simulink model "PMSM_Simulation_2025a"  (R2025a)
settings: Solver=FixedStepDiscrete  StartTime=0.0  StopTime=10  FixedStep=0.00005/200  RelTol=1e-3
values from neighbouring files (symbols this model uses):
  MC_DCurrLopKi_CFG = 0.008293758    [PMSM_MC_Data_2025a.sldd]
  MC_DCurrLopKp_CFG = 0.0870848    [PMSM_MC_Data_2025a.sldd]
  MC_MotModeDebug_CFG = 255.0    [PMSM_MC_Data_2025a.sldd]
  MC_POLE_NUM_CFG = 7.0    [PMSM_MC_Data_2025a.sldd]
  MC_QCurrLopKi_CFG = 0.008293758    [PMSM_MC_Data_2025a.sldd]
  MC_QCurrLopKp_CFG = 0.0870848    [PMSM_MC_Data_2025a.sldd]
  MC_SpdLopKi_CFG = 1.0E-5    [PMSM_MC_Data_2025a.sldd]
  MC_SpdLopKp_CFG = 0.002    [PMSM_MC_Data_2025a.sldd]
undefined symbols (not defined in the file or in its folder): Ls, magnitude, Rs
libraries: simulink x28, slpidlib x6, spsDCVoltageSourceLib x1, spsPermanentMagnetSynchronousMachineLib x1, spsUniversalBridgeLib x1, sps_lib x1
(part 2 of 3)

== system PMSM_Simulation_2025a/PMSM_MC/MC_HighFrqTask/FOC/SensorLessAlgorithm ==
  note: MotorSpdRef用于
      | 方向极性判定使用
  MotorSpdRef : Inport
  Ialpha : Inport  Port=2
  Ibeta : Inport  Port=3
  Ualpha : Inport  Port=4
  Ubeta : Inport  Port=5
  Compare To Constant : simulink/Logic and Bit Operations/Compare To Constant  relop===  const=0  OutDataTypeStr=boolean
  Compare To Constant1 : simulink/Logic and Bit Operations/Compare To Constant  relop===  const=1  OutDataTypeStr=boolean
  Compare To Constant2 : simulink/Logic and Bit Operations/Compare To Constant  relop===  const=2  OutDataTypeStr=boolean
  Compare To Constant3 : simulink/Logic and Bit Operations/Compare To Constant  relop===  const=3  OutDataTypeStr=boolean
  Constant : Constant  Value=uint8(3)
  FluxObs+PLL : Subsystem
  Luenberger+PLL : Subsystem
  Merge : Merge  Inputs=4
  Merge1 : Merge  Inputs=4
  SMO+Artan : Subsystem
  SMO+PLL : Subsystem
  Thetae_Est : Outport
  We_Est : Outport  Port=2
  wires:
  MotorSpdRef/1 -> SMO+Artan/1(MotorSpdRef), Luenberger+PLL/1(MotorSpdRef), FluxObs+PLL/1(MotorSpdRef), SMO+PLL/1(MotorSpdRef)
  Ialpha/1 -> SMO+Artan/2(Ialpha), Luenberger+PLL/2(Ialpha), FluxObs+PLL/2(Ialpha), SMO+PLL/2(Ialpha)
  Ibeta/1 -> Luenberger+PLL/3(Ibeta), FluxObs+PLL/3(Ibeta), SMO+PLL/3(Ibeta), SMO+Artan/3(Ibeta)
  Ualpha/1 -> Luenberger+PLL/4(Ualpha), FluxObs+PLL/4(Ualpha), SMO+PLL/4(Ualpha), SMO+Artan/4(Ualpha)
  Ubeta/1 -> Luenberger+PLL/5(Ubeta), FluxObs+PLL/5(Ubeta), SMO+PLL/5(Ubeta), SMO+Artan/5(Ubeta)
  Constant/1 -> Compare To Constant3/1, Compare To Constant2/1, Compare To Constant1/1, Compare To Constant/1
  Compare To Constant/1 -> SMO+Artan/Enable
  Compare To Constant1/1 -> SMO+PLL/Enable
  Compare To Constant2/1 -> FluxObs+PLL/Enable
  SMO+Artan/1(Thetae_Est) -> Merge/1
  SMO+PLL/1(Thetae_Est) -> Merge/2
  FluxObs+PLL/1(Thetae_Est) -> Merge/3
  Luenberger+PLL/1(Thetae_Est) -> Merge/4
  SMO+Artan/2(We_Est) -> Merge1/1
  SMO+PLL/2(We_Est) -> Merge1/2
  FluxObs+PLL/2(We_Est) -> Merge1/3
  Luenberger+PLL/2(We_Est) -> Merge1/4
  Merge1/1 -> We_Est/1
  Merge/1 -> Thetae_Est/1
  Compare To Constant3/1 -> Luenberger+PLL/Enable

== system PMSM_Simulation_2025a/PMSM_MC/MC_HighFrqTask/OpenLopMod/AngleNormalization ==
  note: 用于将观测器估算的输入角度归一化到[0 2pi]的角度输出
  Theta : Inport
  Abs : Abs  SaturateOnIntegerOverflow=off
  Add : Sum  Inputs=+-
  Compare To Zero : simulink/Logic and Bit Operations/Compare To Zero  relop=>=  OutDataTypeStr=boolean
  Constant : Constant  Value=single(6.28)
  Constant1 : Constant  Value=single(6.28)
  Constant2 : Constant  Value=single(6.28)
  Mod : Math  Operator=mod
  Mod1 : Math  Operator=mod
  Switch : Switch  Criteria=u2 ~= 0  SaturateOnIntegerOverflow=off  InputSameDT=off
  ThetaNorm : Outport
  wires:
  Theta/1 -> Abs/1, Mod/1, Compare To Zero/1
  Compare To Zero/1 -> Switch/2
  Constant/1 -> Mod/2
  Mod/1 -> Switch/1
  Abs/1 -> Mod1/1
  Constant1/1 -> Mod1/2
  Add/1 -> Switch/3
  Mod1/1 -> Add/2
  Constant2/1 -> Add/1
  Switch/1 -> ThetaNorm/1

== system PMSM_Simulation_2025a/PMSM_MC/MC_LowFrqTask/MotSpdCal/LPF ==
  In : Inport
  TiCon : Inport  Port=2
  Add : Sum  Inputs=+-
  Add1 : Sum
  Constant : Constant  Value=single(1)
  Delay : Delay  DelayLength=1  InitialConditionSource=Input port
      settings: InputPortMap=u0,p4
  Product : Product
  Product1 : Product
  out : Outport
  wires:
  In/1 -> Delay/2, Product/1
  TiCon/1 -> Add/2, Product/2
  Add/1 -> Product1/1
  Constant/1 -> Add/1
  Product/1 -> Add1/1
  Product1/1 -> Add1/2
  Add1/1 -> Delay/1, out/1
  Delay/1 -> Product1/2

== system PMSM_Simulation_2025a/PMSM_MC/MC_LowFrqTask/MotSpdCal/LPF1 ==
  In : Inport
  TiCon : Inport  Port=2
  Add : Sum  Inputs=+-
  Add1 : Sum
  Constant : Constant  Value=single(1)
  Delay : Delay  DelayLength=1  InitialConditionSource=Input port
      settings: InputPortMap=u0,p4
  Product : Product
  Product1 : Product
  out : Outport
  wires:
  In/1 -> Delay/2, Product/1
  TiCon/1 -> Add/2, Product/2
  Add/1 -> Product1/1
  Constant/1 -> Add/1
  Product/1 -> Add1/1
  Product1/1 -> Add1/2
  Add1/1 -> Delay/1, out/1
  Delay/1 -> Product1/2

== system PMSM_Simulation_2025a/PMSM_MC/MC_HighFrqTask/ElecAngleCal/AngleCal/If Action Subsystem ==
  Ecode_PhyVal : Inport
  Action Port : ActionPort  ActionPortLabel=if(u1 == 1)
  Constant : Constant  Value=MC_POLE_NUM_CFG
  Constant1 : Constant  Value=int32(16384)
  Constant2 : Constant  Value=int32(16384)
  Constant3 : Constant  Value=single(6.28)
  Data Type Conversion : DataTypeConversion  OutDataTypeStr=single  SaturateOnIntegerOverflow=off  RndMeth=Floor
  Data Type Conversion1 : DataTypeConversion  OutDataTypeStr=single  SaturateOnIntegerOverflow=off  RndMeth=Floor
  Data Type Conversion2 : DataTypeConversion  OutDataTypeStr=single  SaturateOnIntegerOverflow=off  RndMeth=Floor
  Divide : Product  Inputs=*/
  Mod : Math  Operator=mod
  Mux : Mux  Inputs=2
  Product : Product
  Product1 : Product
  Out1 : Outport
  wires:
  Ecode_PhyVal/1 -> Mod/1
  Constant1/1 -> Mod/2
  Mod/1 -> Data Type Conversion/1
  Data Type Conversion/1 -> Divide/1
  Constant2/1 -> Divide/2
  Divide/1 -> Product/1
  Constant3/1 -> Product/2
  Constant/1 -> Data Type Conversion1/1
  Data Type Conversion1/1 -> Product1/2
  Product/1 -> Product1/1, Mux/1
  Product1/1 -> Data Type Conversion2/1
  Data Type Conversion2/1 -> Mux/2
  Mux/1 -> Out1/1

== system PMSM_Simulation_2025a/PMSM_MC/MC_HighFrqTask/ElecAngleCal/AngleCal/If Action Subsystem1 ==
  Ecode_PhyVal : Inport
  Action Port : ActionPort  ActionPortLabel=elseif(u1 == -1)
  Constant : Constant  Value=MC_POLE_NUM_CFG
  Constant1 : Constant  Value=int32(16384)
  Constant2 : Constant  Value=int32(16384)
  Constant3 : Constant  Value=single(6.28)
  Data Type Conversion : DataTypeConversion  OutDataTypeStr=single  SaturateOnIntegerOverflow=off  RndMeth=Floor
  Data Type Conversion1 : DataTypeConversion  OutDataTypeStr=single  SaturateOnIntegerOverflow=off  RndMeth=Floor
  Data Type Conversion2 : DataTypeConversion  OutDataTypeStr=single  SaturateOnIntegerOverflow=off  RndMeth=Floor
  Data Type Conversion3 : DataTypeConversion  OutDataTypeStr=int32  SaturateOnIntegerOverflow=off  RndMeth=Floor
  Divide : Product  Inputs=*/
  Gain : Gain  Gain=-1
  Gain1 : Gain  Gain=-1
  Mod : Math  Operator=mod
  Mux : Mux  Inputs=2
  Product : Product
  Product1 : Product
  Out1 : Outport
  wires:
  Constant1/1 -> Mod/2
  Mod/1 -> Data Type Conversion/1
  Constant2/1 -> Divide/2
  Constant3/1 -> Product/2
  Data Type Conversion2/1 -> Mux/2
  Product/1 -> Product1/1, Mux/1
  Divide/1 -> Product/1
  Constant/1 -> Data Type Conversion1/1
  Data Type Conversion/1 -> Divide/1
  Product1/1 -> Data Type Conversion2/1
  Data Type Conversion1/1 -> Product1/2
  Ecode_PhyVal/1 -> Gain/1
  Gain/1 -> Data Type Conversion3/1
  Data Type Conversion3/1 -> Mod/1
  Mux/1 -> Gain1/1
  Gain1/1 -> Out1/1

== system PMSM_Simulation_2025a/PMSM_MC/MC_HighFrqTask/ElecAngleCal/AngleCal/If Action Subsystem2 ==
  Action Port : ActionPort  ActionPortLabel=else
  Constant : Constant  Value=single(0)
  Constant1 : Constant  Value=single(0)
  Mux : Mux  Inputs=2
  Out1 : Outport
  wires:
  Constant/1 -> Mux/1
  Constant1/1 -> Mux/2
  Mux/1 -> Out1/1

== system PMSM_Simulation_2025a/PMSM_MC/MC_HighFrqTask/FOC/SVPWM/SevenSegSVPWM ==
  Uα : Inport
  Uβ : Inport  Port=2
  VBus : Inport  Port=3
  Demux : Demux  Outputs=3
  SectorCaculate : Subsystem
  T1T2Caculate : Subsystem
  TcmCaculate : Subsystem
  Tpwm : Constant  Value=single(1)
  XYZCaculate : Subsystem
  UVoltage_PWM : Outport
  VVoltage_PWM : Outport  Port=2
  WVoltage_PWM : Outport  Port=3
  wires:
  Uα/1 -> SectorCaculate/1(Ualpha), XYZCaculate/1(Ualpha)
  Uβ/1 -> XYZCaculate/2(Ubeta), SectorCaculate/2(Ubeta)
  VBus/1 -> XYZCaculate/3(Udc)
  Tpwm/1 -> TcmCaculate/4(Tpwm), T1T2Caculate/3(Tpwm), XYZCaculate/4(Ts)
  SectorCaculate/1(N) -> TcmCaculate/1(N), T1T2Caculate/1(N)
  XYZCaculate/1(XYZ) -> T1T2Caculate/2(XYZ)
  T1T2Caculate/1(T1) -> TcmCaculate/2(T1)
  T1T2Caculate/2(T2) -> TcmCaculate/3(T2)
  TcmCaculate/1(Tcm1 Tcm2 Tcm3) -> Demux/1
  Demux/1 -> UVoltage_PWM/1
  Demux/2 -> VVoltage_PWM/1
  Demux/3 -> WVoltage_PWM/1

== system PMSM_Simulation_2025a/PMSM_MC/MC_HighFrqTask/FOC/SensorLessAlgorithm/FluxObs+PLL ==
  MotorSpdRef : Inport
  Ialpha : Inport  Port=2
  Ibeta : Inport  Port=3
  Ualpha : Inport  Port=4
  Ubeta : Inport  Port=5
  Enable : EnablePort
  FluxObs : Subsystem
  PLL : Subsystem
  Thetae_Est : Outport
  We_Est : Outport  Port=2
  wires:
  Ubeta/1 -> FluxObs/4(Ubeta)
  Ualpha/1 -> FluxObs/3(Ualpha)
  Ialpha/1 -> FluxObs/1(Ialpha)
  Ibeta/1 -> FluxObs/2(Ibeta)
  PLL/1(Thetae_Est) -> Thetae_Est/1
  PLL/2(We_Est) -> We_Est/1
  FluxObs/2(Flux_beta) -> PLL/3(Flux_beta)
  FluxObs/1(Flux_alpha) -> PLL/2(Flux_alpha)
  MotorSpdRef/1 -> PLL/1(MotorSpdRef)

== system PMSM_Simulation_2025a/PMSM_MC/MC_HighFrqTask/FOC/SensorLessAlgorithm/Luenberger+PLL ==
  MotorSpdRef : Inport
  Ialpha : Inport  Port=2
  Ibeta : Inport  Port=3
  Ualpha : Inport  Port=4
  Ubeta : Inport  Port=5
  Enable : EnablePort
  Delay : Delay  DelayLength=1
  Luenberger : Subsystem
  PLL : Subsystem
  Thetae_Est : Outport
  We_Est : Outport  Port=2
  wires:
  MotorSpdRef/1 -> PLL/1(MotorSpdRef)
  Luenberger/1(AlphaE) -> PLL/2(AlphaE)
  Luenberger/2(BetaE) -> PLL/3(BetaE)
  PLL/2(We_Est) -> Delay/1, We_Est/1
  PLL/1(Thetae_Est) -> Thetae_Est/1
  Ibeta/1 -> Luenberger/2(Ibeta)
  Ialpha/1 -> Luenberger/1(Ialpha)
  Ualpha/1 -> Luenberger/3(Ualpha)
  Ubeta/1 -> Luenberger/4(Ubeta)
  Delay/1 -> Luenberger/5(We)

== system PMSM_Simulation_2025a/PMSM_MC/MC_HighFrqTask/FOC/SensorLessAlgorithm/SMO+Artan ==
  MotorSpdRef : Inport
  Ialpha : Inport  Port=2
  Ibeta : Inport  Port=3
  Ualpha : Inport  Port=4
  Ubeta : Inport  Port=5
  Enable : EnablePort
  Artan : Subsystem
  SMO : Subsystem
  Thetae_Est : Outport
  We_Est : Outport  Port=2
  wires:
  Ialpha/1 -> SMO/1(Ialpha)
  Ibeta/1 -> SMO/2(Ibeta)
  Ualpha/1 -> SMO/3(Ualpha)
  Ubeta/1 -> SMO/4(Ubeta)
  MotorSpdRef/1 -> Artan/1(MotorSpdRef)
  SMO/1(AlphaE) -> Artan/2(AlphaE)
  SMO/2(BetaE) -> Artan/3(BetaE)
  Artan/2(We_Est) -> We_Est/1
  Artan/1(Thetae_Est) -> Thetae_Est/1

== system PMSM_Simulation_2025a/PMSM_MC/MC_HighFrqTask/FOC/SensorLessAlgorithm/SMO+PLL ==
  MotorSpdRef : Inport
  Ialpha : Inport  Port=2
  Ibeta : Inport  Port=3
  Ualpha : Inport  Port=4
  Ubeta : Inport  Port=5
  Enable : EnablePort
  PLL : Subsystem
  SMO : Subsystem
  Thetae_Est : Outport
  We_Est : Outport  Port=2
  wires:
  MotorSpdRef/1 -> PLL/1(MotorSpdRef)
  SMO/1(AlphaE) -> PLL/2(AlphaE)
  SMO/2(BetaE) -> PLL/3(BetaE)
  PLL/2(We_Est) -> We_Est/1
  PLL/1(Thetae_Est) -> Thetae_Est/1
  Ibeta/1 -> SMO/2(Ibeta)
  Ialpha/1 -> SMO/1(Ialpha)
  Ualpha/1 -> SMO/3(Ualpha)
  Ubeta/1 -> SMO/4(Ubeta)

== system PMSM_Simulation_2025a/PMSM_MC/MC_HighFrqTask/FOC/SVPWM/SevenSegSVPWM/SectorCaculate ==
  Ualpha : Inport
  Ubeta : Inport  Port=2
  A : Fcn  Expr=u[2]
  Add : Sum  Inputs=+++
  B : Fcn  Expr=u(1)*sqrt(3/4)-0.5*u[2]
  C : Fcn  Expr=-u[1]*sqrt(3/4)-u[2]*0.5
  Constant : Constant  Value=uint8(1)
  Constant1 : Constant  Value=uint8(0)
  Data Type Conversion : DataTypeConversion  OutDataTypeStr=uint8  SaturateOnIntegerOverflow=off  RndMeth=Floor
  Gain : Gain  Gain=2
  Gain1 : Gain  Gain=4
  Mux : Mux  Inputs=2
  Switch : Switch  Criteria=u2 > Threshold  SaturateOnIntegerOverflow=off  InputSameDT=off
  Switch1 : Switch  Criteria=u2 > Threshold  SaturateOnIntegerOverflow=off  InputSameDT=off
  Switch2 : Switch  Criteria=u2 > Threshold  SaturateOnIntegerOverflow=off  InputSameDT=off
  N : Outport
  wires:
  Ualpha/1 -> Mux/1
  Ubeta/1 -> Mux/2
  Mux/1 -> C/1, A/1, B/1
  A/1 -> Switch/2
  B/1 -> Switch1/2
  C/1 -> Switch2/2
  Constant/1 -> Switch/1, Switch2/1, Switch1/1
  Constant1/1 -> Switch/3, Switch1/3, Switch2/3
  Switch2/1 -> Gain1/1
  Switch1/1 -> Gain/1
  Gain/1 -> Add/2
  Gain1/1 -> Add/3
  Switch/1 -> Add/1
  Add/1 -> Data Type Conversion/1
  Data Type Conversion/1 -> N/1

== system PMSM_Simulation_2025a/PMSM_MC/MC_HighFrqTask/FOC/SVPWM/SevenSegSVPWM/T1T2Caculate ==
  N : Inport
  XYZ : Inport  Port=2
  Tpwm : Inport  Port=3
  Abs : Abs  SaturateOnIntegerOverflow=off
  Abs1 : Abs  SaturateOnIntegerOverflow=off
  Demux : Demux  Outputs=3
  Fcn : Fcn  Expr=u(1)*u(3)/(u(1)+u(2))
  Fcn1 : Fcn  Expr=u(2)*u(3)/(u(1)+u(2))
  Fcn2 : Fcn  Expr=u(3)-u(2)-u(1)
  Gain : Gain  Gain=-1
  Gain1 : Gain  Gain=-1
  Gain2 : Gain  Gain=-1
  Multiport Switch : MultiPortSwitch  Inputs=6  DiagnosticForDefault=None  SaturateOnIntegerOverflow=off  InputSameDT=off
  Multiport Switch1 : MultiPortSwitch  Inputs=6  DiagnosticForDefault=None  SaturateOnIntegerOverflow=off  InputSameDT=off
  Mux : Mux  Inputs=3
  Switch : Switch  SaturateOnIntegerOverflow=off  InputSameDT=off
  Switch1 : Switch  SaturateOnIntegerOverflow=off  InputSameDT=off
  T1 : Outport
  T2 : Outport  Port=2
  wires:
  N/1 -> Multiport Switch/1, Multiport Switch1/1
  XYZ/1 -> Demux/1
  Demux/1 -> Gain/1, Multiport Switch/6, Multiport Switch1/4
  Demux/2 -> Gain1/1, Multiport Switch/3, Multiport Switch1/2
  Demux/3 -> Gain2/1, Multiport Switch1/5, Multiport Switch/2
  Gain/1 -> Multiport Switch1/3, Multiport Switch/5
  Gain2/1 -> Multiport Switch1/7, Multiport Switch/4
  Gain1/1 -> Multiport Switch/7, Multiport Switch1/6
  Multiport Switch/1 -> Switch/1, Mux/1  "T1"
  Multiport Switch1/1 -> Switch1/1, Mux/2  "T2"
  Tpwm/1 -> Mux/3
  Mux/1 -> Fcn1/1, Fcn/1, Fcn2/1
  Fcn/1 -> Switch/3
  Fcn1/1 -> Switch1/3
  Fcn2/1 -> Switch1/2, Switch/2
  Switch/1 -> Abs/1
  Abs/1 -> T1/1
  Switch1/1 -> Abs1/1
  Abs1/1 -> T2/1

== system PMSM_Simulation_2025a/PMSM_MC/MC_HighFrqTask/FOC/SVPWM/SevenSegSVPWM/TcmCaculate ==
  N : Inport
  T1 : Inport  Port=2
  T2 : Inport  Port=3
  Tpwm : Inport  Port=4
  Fcn : Fcn  Expr=(u(3)+u(1)+u(2))/2
  Fcn1 : Fcn  Expr=(u(3)-u(1)+u(2))/2
  Fcn2 : Fcn  Expr=(u(3)-u(1)-u(2))/2
  Multiport Switch : MultiPortSwitch  Inputs=6  DiagnosticForDefault=None  SaturateOnIntegerOverflow=off  InputSameDT=off
  Multiport Switch1 : MultiPortSwitch  Inputs=6  DiagnosticForDefault=None  SaturateOnIntegerOverflow=off  InputSameDT=off
  Multiport Switch2 : MultiPortSwitch  Inputs=6  DiagnosticForDefault=None  SaturateOnIntegerOverflow=off  InputSameDT=off
  Mux : Mux  Inputs=3
  Mux1 : Mux  Inputs=3
  Tcm1 Tcm2 Tcm3 : Outport
  wires:
  Mux/1 -> Tcm1 Tcm2 Tcm3/1
  T2/1 -> Mux1/2
  T1/1 -> Mux1/1
  Tpwm/1 -> Mux1/3
  Mux1/1 -> Fcn/1, Fcn2/1, Fcn1/1
  N/1 -> Multiport Switch2/1, Multiport Switch1/1, Multiport Switch/1
  Fcn1/1 -> Multiport Switch1/4, Multiport Switch/7, Multiport Switch/2, Multiport Switch1/5, Multiport Switch2/6, Multiport Switch2/3
  Fcn/1 -> Multiport Switch1/6, Multiport Switch2/7, Multiport Switch2/5, Multiport Switch/4, Multiport Switch/3, Multiport Switch1/2
  Fcn2/1 -> Multiport Switch1/7, Multiport Switch/6, Multiport Switch/5, Multiport Switch1/3, Multiport Switch2/4, Multiport Switch2/2
  Multiport Switch/1 -> Mux/1
  Multiport Switch1/1 -> Mux/2
  Multiport Switch2/1 -> Mux/3

== system PMSM_Simulation_2025a/PMSM_MC/MC_HighFrqTask/FOC/SVPWM/SevenSegSVPWM/XYZCaculate ==
  Ualpha : Inport
  Ubeta : Inport  Port=2
  Udc : Inport  Port=3
  Ts : Inport  Port=4
  Add : Sum
  Add1 : Sum  Inputs=+-
  Fcn : Fcn  Expr=1/u
  Gain : Gain  Gain=3/2
  Gain1 : Gain  Gain=sqrt(3)
  Gain2 : Gain  Gain=sqrt(3)/2
  Mux : Mux  Inputs=3
  Product{,1..3} (4 alike) : Product
  XYZ : Outport
  wires:
  Ualpha/1 -> Gain/1
  Ubeta/1 -> Gain2/1, Gain1/1
  Gain/1 -> Add/2, Add1/2
  Gain1/1 -> Product/1
  Gain2/1 -> Add1/1, Add/1
  Ts/1 -> Product3/1
  Product3/1 -> Product1/2, Product/2, Product2/2
  Add/1 -> Product1/1
  Udc/1 -> Fcn/1
  Fcn/1 -> Product3/2
  Add1/1 -> Product2/1
  Product1/1 -> Mux/2
  Product2/1 -> Mux/3
  Product/1 -> Mux/1
  Mux/1 -> XYZ/1

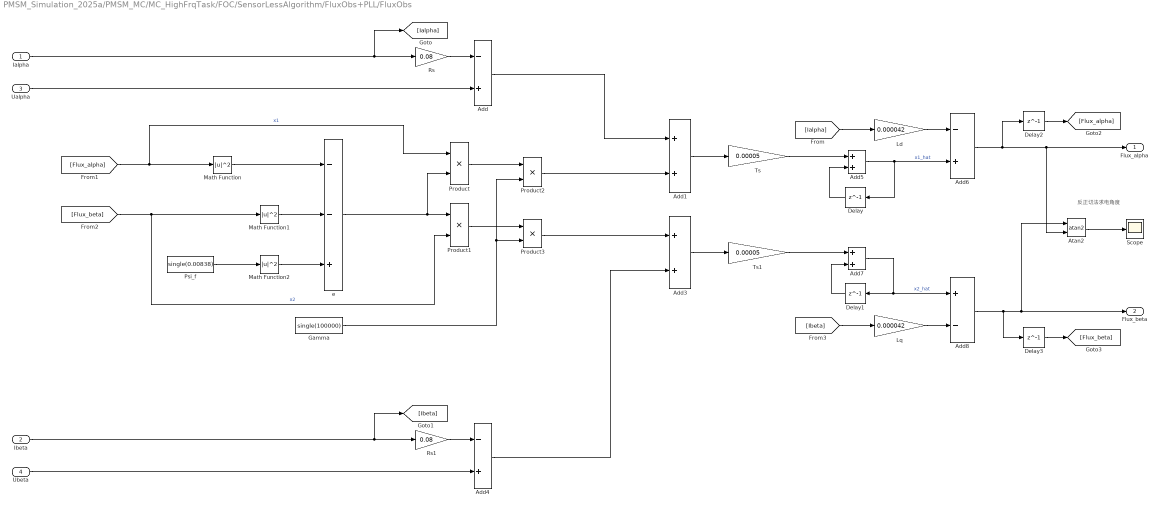
== system PMSM_Simulation_2025a/PMSM_MC/MC_HighFrqTask/FOC/SensorLessAlgorithm/FluxObs+PLL/FluxObs ==
  note: 反正切法求电角度
  Ialpha : Inport
  Ibeta : Inport  Port=2
  Ualpha : Inport  Port=3
  Ubeta : Inport  Port=4
  Add : Sum  Inputs=-+
  Add{1,3,5,7} (4 alike) : Sum
  Add4 : Sum  Inputs=-+
  Add6 : Sum  Inputs=-+
  Add8 : Sum  Inputs=+-
  Atan2 : Trigonometry  Operator=atan2
  Delay{,1..3} (4 alike) : Delay  DelayLength=1
  Gamma : Constant  Value=single(100000)
  Ld : Gain  Gain=0.000042
  Lq : Gain  Gain=0.000042
  Math Function : Math  Operator=magnitude^2
  Math Function1 : Math  Operator=magnitude^2
  Math Function2 : Math  Operator=magnitude^2
  Product{,1..3} (4 alike) : Product
  Psi_f : Constant  Value=single(0.00838)
  Rs : Gain  Gain=0.08
  Rs1 : Gain  Gain=0.08
  Scope : Scope
      settings: ActiveDisplayYMinimum=-3.9256648123264313  ActiveDisplayYMaximum=3.9258014261722565  DataLoggingVariableName=ScopeData8
  Ts : Gain  Gain=0.00005
  Ts1 : Gain  Gain=0.00005
  e : Sum  Inputs=--+
  Flux_alpha : Outport
  Flux_beta : Outport  Port=2
  wires:
  Ialpha/1 -> [Ialpha], Rs/1
  Rs/1 -> Add/1
  Ualpha/1 -> Add/2
  Add/1 -> Add1/1
  [Flux_alpha] -> Product/1, Math Function/1  "x1"
  Math Function/1 -> e/1
  [Flux_beta] -> Product1/2, Math Function1/1  "x2"
  Math Function1/1 -> e/2
  Math Function2/1 -> e/3
  Psi_f/1 -> Math Function2/1
  e/1 -> Product1/1, Product/2
  Product/1 -> Product2/1
  Product1/1 -> Product3/1
  Gamma/1 -> Product2/2, Product3/2
  Product2/1 -> Add1/2
  Product3/1 -> Add3/1
  Ubeta/1 -> Add4/2
  Ibeta/1 -> [Ibeta], Rs1/1
  Rs1/1 -> Add4/1
  Add4/1 -> Add3/2
  Add1/1 -> Ts/1
  Add3/1 -> Ts1/1
  Ts/1 -> Add5/1
  [Ialpha] -> Ld/1
  Ld/1 -> Add6/1
  Add5/1 -> Delay/1, Add6/2  "x1_hat"
  Delay/1 -> Add5/2
  Ts1/1 -> Add7/1
  Add7/1 -> Add8/1, Delay1/1  "x2_hat"
  Delay1/1 -> Add7/2
  Lq/1 -> Add8/2
  [Ibeta] -> Lq/1
  Add6/1 -> Delay2/1, Atan2/2, Flux_alpha/1
  Add8/1 -> Delay3/1, Atan2/1, Flux_beta/1
  Delay2/1 -> [Flux_alpha]
  Delay3/1 -> [Flux_beta]
  Atan2/1 -> Scope/1

== system PMSM_Simulation_2025a/PMSM_MC/MC_HighFrqTask/FOC/SensorLessAlgorithm/FluxObs+PLL/PLL ==
  MotorSpdRef : Inport
  Flux_alpha : Inport  Port=2
  Flux_beta : Inport  Port=3
  Add : Sum
  Constant : Constant  Value=single(52000)
  Constant1 : Constant  Value=single(0.0085)
  Constant4 : Constant  Value=single(40)
  Constant5 : Constant  Value=single(2*pi)
  Cos : Trigonometry  Operator=cos
  Delay : Delay  DelayLength=1
  Gain : Gain  Gain=0.00005
  LPF : Subsystem
  Mod : Math  Operator=mod
  PI_Out : Scope  NumInputPorts=2
      settings: ActiveDisplayYMinimum=-82.912358522415147  ActiveDisplayYMaximum=519.20902562141418  DataLoggingVariableName=ScopeData11
  PLL_PI : slpidlib/PID Controller  Controller=PI  Form=Parallel  TimeDomain=Discrete-time  UseExternalTs=off  SampleTime=-1  IntegratorMethod=Forward Euler  FilterMethod=Forward Euler  ControllerParametersSource=external  P=1  I=1  UseKiTs=on  D=0  UseExternalDerivativeSource=off  N=100  UseFilter=on  TunerSelectOption=Transfer Function Based (PID Tuner App)  InitialConditionSource=internal  InitialConditionForIntegrator=0  InitialConditionForFilter=0  DifferentiatorICPrevScaledInput=0  ExternalReset=none  TrackingMode=off  Kt=1  LimitOutput=off  SatLimitsSource=internal  UpperSaturationLimit=inf  LowerSaturationLimit=-inf  LinearizeAsGain=off  AntiWindupMode=none  Kb=1  LimitIntegrator=off  UpperIntegratorSaturationLimit=8000  LowerIntegratorSaturationLimit=-8000  POutMin=[]  POutMax=[]  IOutMin=[]  IOutMax=[]  DOutMin=[]  DOutMax=[]  NOutMin=[]  NOutMax=[]  SumOutMin=[]  SumOutMax=[]  SaturationOutMin=[]  SaturationOutMax=[]  PParamMin=[]  PParamMax=[]  IParamMin=[]  IParamMax=[]  DParamMin=[]  DParamMax=[]  NParamMin=[]  NParamMax=[]  KbParamMin=[]  KbParamMax=[]  KtParamMin=[]  KtParamMax=[]  KbOutMin=[]  KbOutMax=[]  KtOutMin=[]  KtOutMax=[]  IntegratorOutMin=[]  IntegratorOutMax=[]  FilterOutMin=[]  FilterOutMax=[]  SumI1OutMin=[]  SumI1OutMax=[]  SumI2OutMin=[]  SumI2OutMax=[]  SumI3OutMin=[]  SumI3OutMax=[]  SumI4OutMin=[]  SumI4OutMax=[]  SumDOutMin=[]  SumDOutMax=[]  DifferentiatorOutMin=[]  DifferentiatorOutMax=[]  FilterDiffOutCoefMin=[]  FilterDiffOutCoefMax=[]  ReciprocalOutMin=[]  ReciprocalOutMax=[]  SumDenOutMin=[]  SumDenOutMax=[]  SumNumOutMin=[]  SumNumOutMax=[]  DivideOutMin=[]  DivideOutMax=[]  UdiffTsProdOutMin=[]  UdiffTsProdOutMax=[]  NTsProdOutMin=[]  NTsProdOutMax=[]  UintegralTsProdOutMin=[]  UintegralTsProdOutMax=[]  UngainTsProdOutMin=[]  UngainTsProdOutMax=[]  ClampingZeroOutDataTypeStr=Inherit: Inherit via back propagation  ClampingZeroOutMin=[]  ClampingZeroOutMax=[]  FilterDenConstantOutDataTypeStr=Inherit: Inherit via back propagation  FilterDenConstantOutMin=[]  FilterDenConstantOutMax=[]  PCopyOutDataTypeStr=Inherit: Inherit via back propagation  PCopyOutMin=[]  PCopyOutMax=[]  NCopyOutDataTypeStr=Inherit: Inherit via back propagation  NCopyOutMin=[]  NCopyOutMax=[]  IntegratorContinuousStateAttributes=''  IntegratorStateMustResolveToSignalObject=off  IntegratorRTWStateStorageClass=Auto  FilterContinuousStateAttributes=''  FilterStateMustResolveToSignalObject=off  FilterRTWStateStorageClass=Auto  ParallelPVariant=ExternalParameters  IdealPVariant=Disabled  IVariant=ExternalParameters  DVariant=Disabled  IntegratorVariant=Discrete  SatVariant=Disabled  AWVariant=Passthrough  PCopyVariant=Disabled  TRVariant=Disabled  FdbkBlocksVariant=Forward  IdealPFdbkVariant=Disabled  SatFdbkVariant=Disabled  DerivativeFilterVariant=Disabled  NVariant=Disabled  NCopyVariant=Disabled_SignalSpec  FilterICVariant=Disabled  IntegratorICVariant=InternalICs  ExternalResetVariant=Disabled  TRSumVariant=Passthrough  SumFdbkVariant=Disabled  SumVariant=Sum_PI  TsampFilterVariant=InternalTs  TsampNgainVariant=Passthrough  TsampIntegralVariant=Disabled_SignalSpec  ExternalSaturationOutDataTypeStr=Inherit: Same as second input  DerivativeSourceVariant=Disabled  PreIntVariant=InternalPreInt
      settings: LibrarySourceBlock=simulink/Discrete/Discrete PID Controller
  Product : Product
  Product2 : Product
  Sin : Trigonometry
  err : Sum  Inputs=-+
  erro : Scope
      settings: ActiveDisplayYMinimum=-0.010186117957346141  ActiveDisplayYMaximum=0.0015268082497641442  DataLoggingVariableName=ScopeData10
  Thetae_Est : Outport
  We_Est : Outport  Port=2
  wires:
  Delay/1 -> Add/2, Cos/1, Sin/1
  Mod/1 -> Thetae_Est/1, Delay/1
  Constant5/1 -> Mod/2
  Add/1 -> Mod/1
  Gain/1 -> Add/1
  PLL_PI/1 -> PI_Out/1, LPF/1(In), Gain/1
  Constant4/1 -> PLL_PI/3
  Constant/1 -> PLL_PI/2
  Cos/1 -> Product2/1
  Sin/1 -> Product/1
  LPF/1(out) -> PI_Out/2, We_Est/1
  Constant1/1 -> LPF/2(TiCon)
  Flux_alpha/1 -> Product/2
  Flux_beta/1 -> Product2/2
  Product/1 -> err/1
  Product2/1 -> err/2
  err/1 -> erro/1, PLL_PI/1

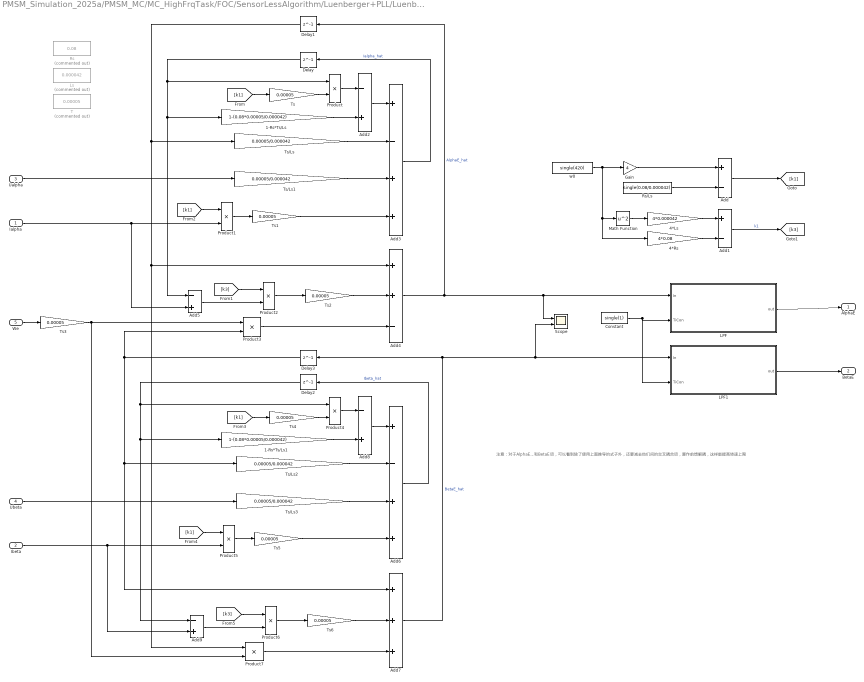
== system PMSM_Simulation_2025a/PMSM_MC/MC_HighFrqTask/FOC/SensorLessAlgorithm/Luenberger+PLL/Luenberger ==
  note: 注意：对于AlphaE和BetaE项，可以看到除了使用上面推导的式子外，还要减去他们间的交叉耦合项，算作前馈解耦，这样能提高转速上限
  Ialpha : Inport
  Ibeta : Inport  Port=2
  Ualpha : Inport  Port=3
  Ubeta : Inport  Port=4
  We : Inport  Port=5
  1-Rs*Ts/Ls : Gain  Gain=1-(0.08*0.00005/0.000042)
  1-Rs*Ts/Ls1 : Gain  Gain=1-(0.08*0.00005/0.000042)
  4*Ls : Gain  Gain=4*0.000042
  4*Rs : Gain  Gain=4*0.08
  Add : Sum  Inputs=+-
  Add1 : Sum  Inputs=+-
  Add{2,5,8..9} (4 alike) : Sum  Inputs=-+
  Add3 : Sum  Inputs=+-++
  Add4 : Sum  Inputs=++-
  Add6 : Sum  Inputs=+-++
  Add7 : Sum  Inputs=+++
  Constant : Constant  Value=single(1)
  Delay{,1..3} (4 alike) : Delay  DelayLength=1
  Gain : Gain  Gain=4
  LPF : Subsystem
  LPF1 : Subsystem
  Ls : Constant  Commented=on  Value=0.000042
  Math Function : Math  Operator=square
  Product{,1..7} (8 alike) : Product
  Rs : Constant  Commented=on  Value=0.08
  Rs/Ls : Constant  Value=single(0.08/0.000042)
  Scope : Scope  NumInputPorts=2
      settings: ActiveDisplayYMinimum=-21.479682207107544  ActiveDisplayYMaximum=21.825211763381958  DataLoggingVariableName=ScopeData18
  T : Constant  Commented=on  Value=0.00005
  Ts{,1..6} (7 alike) : Gain  Gain=0.00005
  Ts/Ls{,1..3} (4 alike) : Gain  Gain=0.00005/0.000042
  w0 : Constant  Value=single(420)
  AlphaE : Outport
  BetaE : Outport  Port=2
  wires:
  w0/1 -> 4*Rs/1, Math Function/1, Gain/1
  Add/1 -> [k1]
  Rs/Ls/1 -> Add/2
  Gain/1 -> Add/1
  4*Ls/1 -> Add1/1
  4*Rs/1 -> Add1/2
  Math Function/1 -> 4*Ls/1
  Add1/1 -> [k3]  "k1"
  [k1] -> Ts/1
  Ts/1 -> Product/2
  Product/1 -> Add2/1
  1-Rs*Ts/Ls/1 -> Add2/2
  Ts/Ls/1 -> Add3/2
  Add2/1 -> Add3/1
  Ts/Ls1/1 -> Add3/3
  [k1] -> Product1/1
  Product1/1 -> Ts1/1
  Ts1/1 -> Add3/4
  Ialpha/1 -> Add5/2, Product1/2
  Ualpha/1 -> Ts/Ls1/1
  Add3/1 -> Delay/1  "Ialpha_hat"
  Delay/1 -> Add5/1, 1-Rs*Ts/Ls/1, Product/1
  Add4/1 -> Scope/1, LPF/1(In), Delay1/1  "AlphaE_hat"
  Delay1/1 -> Product7/1, Add4/1, Ts/Ls/1
  Ts2/1 -> Add4/2
  Product2/1 -> Ts2/1
  [k3] -> Product2/1
  Add5/1 -> Product2/2
  Constant/1 -> LPF1/2(TiCon), LPF/2(TiCon)
  LPF1/1(out) -> BetaE/1
  LPF/1(out) -> AlphaE/1
  We/1 -> Ts3/1
  Product3/1 -> Add4/3
  Add6/1 -> Delay2/1  "Ibeta_hat"
  Product4/1 -> Add8/1
  Delay2/1 -> Product4/1, 1-Rs*Ts/Ls1/1, Add9/1
  1-Rs*Ts/Ls1/1 -> Add8/2
  Ts4/1 -> Product4/2
  [k1] -> Ts4/1
  Add8/1 -> Add6/1
  [k1] -> Product5/1
  Ibeta/1 -> Product5/2, Add9/2
  Delay3/1 -> Ts/Ls2/1, Add7/1, Product3/2
  Ubeta/1 -> Ts/Ls3/1
  Product5/1 -> Ts5/1
  Ts/Ls3/1 -> Add6/3
  Ts5/1 -> Add6/4
  Ts/Ls2/1 -> Add6/2
  Product7/1 -> Add7/3
  Product6/1 -> Ts6/1
  [k3] -> Product6/1
  Add9/1 -> Product6/2
  Ts3/1 -> Product3/1, Product7/2
  Ts6/1 -> Add7/2
  Add7/1 -> Scope/2, LPF1/1(In), Delay3/1  "BetaE_hat"

== system PMSM_Simulation_2025a/PMSM_MC/MC_HighFrqTask/FOC/SensorLessAlgorithm/Luenberger+PLL/PLL ==
  note: 根据误差式子设定来设定反电动势
      | 符号确保使得PLL形成负反馈
  MotorSpdRef : Inport
  AlphaE : Inport  Port=2
  BetaE : Inport  Port=3
  Add : Sum
  Compare To Zero1 : simulink/Logic and Bit Operations/Compare To Zero  relop=>=  OutDataTypeStr=boolean
  Constant : Constant  Value=single(200)
  Constant1 : Constant  Value=single(0.0085)
  Constant2 : Constant  Value=single(-1)
  Constant3 : Constant  Value=single(1)
  Constant4 : Constant  Value=single(2)
  Constant5 : Constant  Value=single(2*pi)
  Cos : Trigonometry  Operator=cos
  Delay : Delay  DelayLength=1
  Gain : Gain  Gain=0.00005
  LPF : Subsystem
  Mod : Math  Operator=mod
  PLL_PI : slpidlib/PID Controller  Controller=PI  Form=Parallel  TimeDomain=Discrete-time  UseExternalTs=off  SampleTime=-1  IntegratorMethod=Forward Euler  FilterMethod=Forward Euler  ControllerParametersSource=external  P=1  I=1  UseKiTs=on  D=0  UseExternalDerivativeSource=off  N=100  UseFilter=on  TunerSelectOption=Transfer Function Based (PID Tuner App)  InitialConditionSource=internal  InitialConditionForIntegrator=0  InitialConditionForFilter=0  DifferentiatorICPrevScaledInput=0  ExternalReset=none  TrackingMode=off  Kt=1  LimitOutput=off  SatLimitsSource=internal  UpperSaturationLimit=inf  LowerSaturationLimit=-inf  LinearizeAsGain=off  AntiWindupMode=none  Kb=1  LimitIntegrator=off  UpperIntegratorSaturationLimit=inf  LowerIntegratorSaturationLimit=-inf  POutMin=[]  POutMax=[]  IOutMin=[]  IOutMax=[]  DOutMin=[]  DOutMax=[]  NOutMin=[]  NOutMax=[]  SumOutMin=[]  SumOutMax=[]  SaturationOutMin=[]  SaturationOutMax=[]  PParamMin=[]  PParamMax=[]  IParamMin=[]  IParamMax=[]  DParamMin=[]  DParamMax=[]  NParamMin=[]  NParamMax=[]  KbParamMin=[]  KbParamMax=[]  KtParamMin=[]  KtParamMax=[]  KbOutMin=[]  KbOutMax=[]  KtOutMin=[]  KtOutMax=[]  IntegratorOutMin=[]  IntegratorOutMax=[]  FilterOutMin=[]  FilterOutMax=[]  SumI1OutMin=[]  SumI1OutMax=[]  SumI2OutMin=[]  SumI2OutMax=[]  SumI3OutMin=[]  SumI3OutMax=[]  SumI4OutMin=[]  SumI4OutMax=[]  SumDOutMin=[]  SumDOutMax=[]  DifferentiatorOutMin=[]  DifferentiatorOutMax=[]  FilterDiffOutCoefMin=[]  FilterDiffOutCoefMax=[]  ReciprocalOutMin=[]  ReciprocalOutMax=[]  SumDenOutMin=[]  SumDenOutMax=[]  SumNumOutMin=[]  SumNumOutMax=[]  DivideOutMin=[]  DivideOutMax=[]  UdiffTsProdOutMin=[]  UdiffTsProdOutMax=[]  NTsProdOutMin=[]  NTsProdOutMax=[]  UintegralTsProdOutMin=[]  UintegralTsProdOutMax=[]  UngainTsProdOutMin=[]  UngainTsProdOutMax=[]  ClampingZeroOutDataTypeStr=Inherit: Inherit via back propagation  ClampingZeroOutMin=[]  ClampingZeroOutMax=[]  FilterDenConstantOutDataTypeStr=Inherit: Inherit via back propagation  FilterDenConstantOutMin=[]  FilterDenConstantOutMax=[]  PCopyOutDataTypeStr=Inherit: Inherit via back propagation  PCopyOutMin=[]  PCopyOutMax=[]  NCopyOutDataTypeStr=Inherit: Inherit via back propagation  NCopyOutMin=[]  NCopyOutMax=[]  IntegratorContinuousStateAttributes=''  IntegratorStateMustResolveToSignalObject=off  IntegratorRTWStateStorageClass=Auto  FilterContinuousStateAttributes=''  FilterStateMustResolveToSignalObject=off  FilterRTWStateStorageClass=Auto  ParallelPVariant=ExternalParameters  IdealPVariant=Disabled  IVariant=ExternalParameters  DVariant=Disabled  IntegratorVariant=Discrete  SatVariant=Disabled  AWVariant=Passthrough  PCopyVariant=Disabled  TRVariant=Disabled  FdbkBlocksVariant=Forward  IdealPFdbkVariant=Disabled  SatFdbkVariant=Disabled  DerivativeFilterVariant=Disabled  NVariant=Disabled  NCopyVariant=Disabled_SignalSpec  FilterICVariant=Disabled  IntegratorICVariant=InternalICs  ExternalResetVariant=Disabled  TRSumVariant=Passthrough  SumFdbkVariant=Disabled  SumVariant=Sum_PI  TsampFilterVariant=InternalTs  TsampNgainVariant=Passthrough  TsampIntegralVariant=Disabled_SignalSpec  ExternalSaturationOutDataTypeStr=Inherit: Same as second input  DerivativeSourceVariant=Disabled  PreIntVariant=InternalPreInt
      settings: LibrarySourceBlock=simulink/Discrete/Discrete PID Controller
  Product{,1..3} (4 alike) : Product
  Sin : Trigonometry
  Switch1 : Switch  Criteria=u2 ~= 0  SaturateOnIntegerOverflow=off  InputSameDT=off
  err : Sum
  Thetae_Est : Outport
  We_Est : Outport  Port=2
  wires:
  Gain/1 -> Add/1
  Mod/1 -> Delay/1, Thetae_Est/1
  AlphaE/1 -> Product/2
  Constant4/1 -> PLL_PI/3
  Product/1 -> Product1/1
  Constant3/1 -> Switch1/3
  Constant5/1 -> Mod/2
  Switch1/1 -> Product3/2, Product1/2
  Product3/1 -> err/2
  Delay/1 -> Cos/1, Sin/1, Add/2
  err/1 -> PLL_PI/1
  Compare To Zero1/1 -> Switch1/2
  Constant2/1 -> Switch1/1
  PLL_PI/1 -> Gain/1, LPF/1(In)
  Cos/1 -> Product/1
  Sin/1 -> Product2/1
  MotorSpdRef/1 -> Compare To Zero1/1
  BetaE/1 -> Product2/2
  Constant/1 -> PLL_PI/2
  LPF/1(out) -> We_Est/1
  Product1/1 -> err/1
  Constant1/1 -> LPF/2(TiCon)
  Product2/1 -> Product3/1
  Add/1 -> Mod/1

== system PMSM_Simulation_2025a/PMSM_MC/MC_HighFrqTask/FOC/SensorLessAlgorithm/SMO+Artan/Artan ==
  note: 速度计算
      | 包含过零处计算处理
  note: 根据速度期望设定来设定反电动势符号
  note: 得使用atan2，而不是atan，
      | 因为atan函数无法判断象限
      | 输出的值是[-PI,PI]
  note: 将角度归一化到[0,2PI]
  MotorSpdRef : Inport
  AlphaE : Inport  Port=2
  BetaE : Inport  Port=3
  Add : Sum  Inputs=+-
  Compare To Zero : simulink/Logic and Bit Operations/Compare To Zero  relop=>=  OutDataTypeStr=boolean
  Constant : Constant  Value=single(2*pi)
  Constant1 : Constant  Value=single(0.01)
  Data Type Conversion : DataTypeConversion  OutDataTypeStr=single  SaturateOnIntegerOverflow=off  RndMeth=Floor
  Gain : Gain  Gain=-1
  Gain1 : Gain  Gain=-1
  LPF : Subsystem
  Product : Product
  Product1 : Product
  Scope : Scope  NumInputPorts=2
      settings: ActiveDisplayYMinimum=-82058.83984375  ActiveDisplayYMaximum=82039.71484375  DataLoggingVariableName=ScopeData13
  Scope1 : Scope
      settings: ActiveDisplayYMinimum=-0.7852557301521299  ActiveDisplayYMaximum=7.0673015713691711  DataLoggingVariableName=ScopeData15
  Sign : Signum
  Sin : Trigonometry  Operator=atan2
  Switch : Switch  Criteria=u2 ~= 0  SaturateOnIntegerOverflow=off  InputSameDT=off
  WeCal : Subsystem
  Thetae_Est : Outport
  We_Est : Outport  Port=2
  wires:
  MotorSpdRef/1 -> Sign/1
  Sign/1 -> Data Type Conversion/1
  AlphaE/1 -> Product/1
  BetaE/1 -> Product1/1
  Data Type Conversion/1 -> Product1/2, Product/2
  Product/1 -> Sin/1
  Product1/1 -> Sin/2
  Sin/1 -> Gain/1
  Gain/1 -> Gain1/1, Switch/1, Compare To Zero/1
  Compare To Zero/1 -> Switch/2
  Gain1/1 -> Add/2
  Constant/1 -> Add/1
  Add/1 -> Switch/3
  Switch/1 -> WeCal/1(ArTan_theta_est), Scope1/1, Thetae_Est/1
  Constant1/1 -> LPF/2(TiCon)
  WeCal/1(We) -> Scope/1, LPF/1(In)
  LPF/1(out) -> Scope/2, We_Est/1

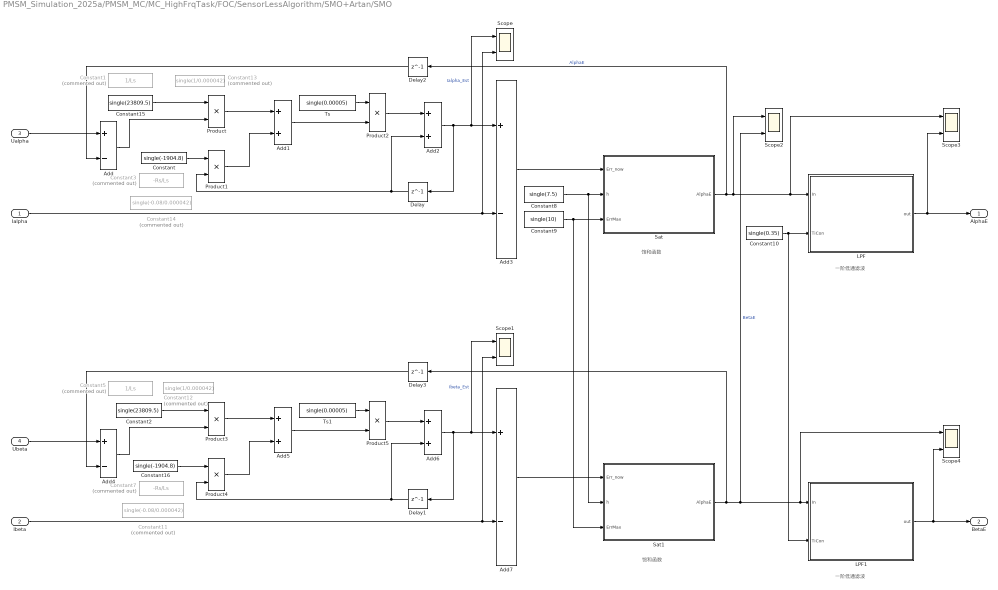
== system PMSM_Simulation_2025a/PMSM_MC/MC_HighFrqTask/FOC/SensorLessAlgorithm/SMO+Artan/SMO ==
  note: 一阶低通滤波
  note: 饱和函数
  note: 饱和函数
  note: 一阶低通滤波
  Ialpha : Inport
  Ibeta : Inport  Port=2
  Ualpha : Inport  Port=3
  Ubeta : Inport  Port=4
  Add{,3..4,7} (4 alike) : Sum  Inputs=+-
  Add{1..2,5..6} (4 alike) : Sum
  Constant : Constant  Value=single(-1904.8)
  Constant1 : Constant  Commented=on  Value=1/Ls
  Constant10 : Constant  Value=single(0.35)
  Constant11 : Constant  Commented=on  Value=single(-0.08/0.000042)
  Constant12 : Constant  Commented=on  Value=single(1/0.000042)
  Constant13 : Constant  Commented=on  Value=single(1/0.000042)
  Constant14 : Constant  Commented=on  Value=single(-0.08/0.000042)
  Constant15 : Constant  Value=single(23809.5)
  Constant16 : Constant  Value=single(-1904.8)
  Constant2 : Constant  Value=single(23809.5)
  Constant3 : Constant  Commented=on  Value=-Rs/Ls
  Constant5 : Constant  Commented=on  Value=1/Ls
  Constant7 : Constant  Commented=on  Value=-Rs/Ls
  Constant8 : Constant  Value=single(7.5)
  Constant9 : Constant  Value=single(10)
  Delay{,1..3} (4 alike) : Delay  DelayLength=1
  LPF : Subsystem
  LPF1 : Subsystem
  Product{,1..5} (6 alike) : Product
  Sat : Subsystem
  Sat1 : Subsystem
  Scope{,1..4} (5 alike) : Scope  NumInputPorts=2
      Scope settings: ActiveDisplayYMinimum=-20.242838406954043  ActiveDisplayYMaximum=19.683035350457061  DataLoggingVariableName=ScopeData2
      Scope1 settings: DataLoggingVariableName=ScopeData3
      Scope2 settings: ActiveDisplayYMinimum=-6.6872910357846731  ActiveDisplayYMaximum=6.6852858453807853  DataLoggingVariableName=ScopeData4
      Scope3 settings: DataLoggingVariableName=ScopeData5
      Scope4 settings: ActiveDisplayYMinimum=-7.4362883952418741  ActiveDisplayYMaximum=7.436170963264396  DataLoggingVariableName=ScopeData6
  Ts : Constant  Value=single(0.00005)
  Ts1 : Constant  Value=single(0.00005)
  AlphaE : Outport
  BetaE : Outport  Port=2
  wires:
  Ualpha/1 -> Add/1
  Constant15/1 -> Product/1
  Add/1 -> Product/2
  Product/1 -> Add1/1
  Constant/1 -> Product1/1
  Product1/1 -> Add1/2
  Add1/1 -> Product2/2
  Ts/1 -> Product2/1
  Product2/1 -> Add2/1
  Add2/1 -> Delay/1, Scope/1, Add3/1  "Ialpha_Est"
  Delay/1 -> Add2/2, Product1/2
  Ialpha/1 -> Scope/2, Add3/2
  Product5/1 -> Add6/1
  Delay1/1 -> Add6/2, Product4/2
  Product3/1 -> Add5/1
  Ibeta/1 -> Scope1/2, Add7/2
  Ts1/1 -> Product5/1
  Add4/1 -> Product3/2
  Constant2/1 -> Product3/1
  Product4/1 -> Add5/2
  Constant16/1 -> Product4/1
  Add5/1 -> Product5/2
  Add6/1 -> Delay1/1, Scope1/1, Add7/1  "Ibeta_Est"
  Ubeta/1 -> Add4/1
  Add3/1 -> Sat/1(Err_now)
  Constant8/1 -> Sat1/2(h), Sat/2(h)
  Constant9/1 -> Sat1/3(ErrMax), Sat/3(ErrMax)
  Add7/1 -> Sat1/1(Err_now)
  Sat/1(AlphaE) -> Scope2/1, Scope3/1, LPF/1(In), Delay2/1  "AlphaE"
  Delay2/1 -> Add/2
  Sat1/1(AlphaE) -> Scope2/2, Scope4/1, LPF1/1(In), Delay3/1  "BetaE"
  Delay3/1 -> Add4/2
  Constant10/1 -> LPF/2(TiCon), LPF1/2(TiCon)
  LPF/1(out) -> Scope3/2, AlphaE/1
  LPF1/1(out) -> Scope4/2, BetaE/1

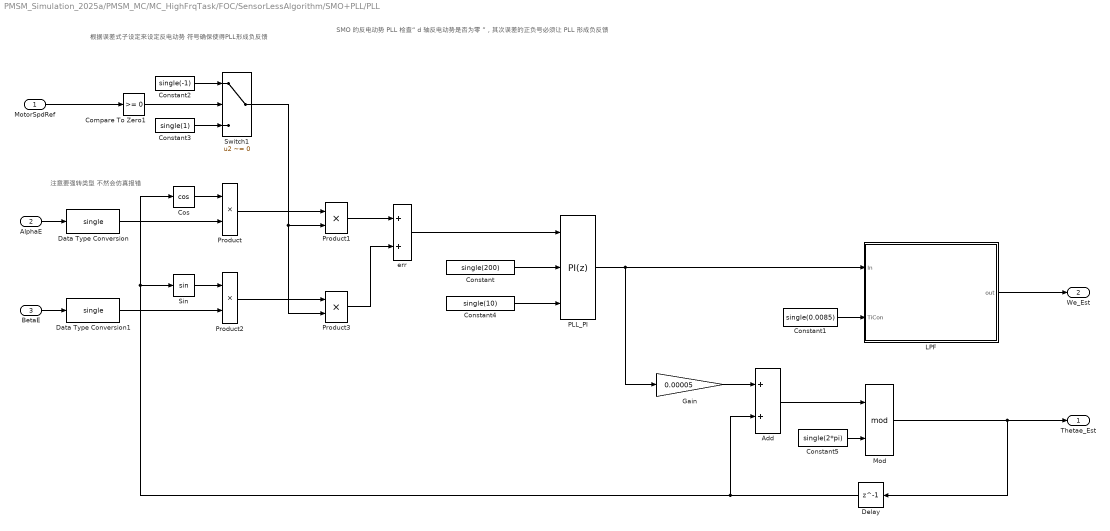
== system PMSM_Simulation_2025a/PMSM_MC/MC_HighFrqTask/FOC/SensorLessAlgorithm/SMO+PLL/PLL ==
  note: SMO 的反电动势 PLL 检查“ d 轴反电动势是否为零 ”，其次误差的正负号必须让 PLL 形成负反馈
  note: 注意要强转类型
      | 不然会仿真报错
  note: 根据误差式子设定来设定反电动势
      | 符号确保使得PLL形成负反馈
  MotorSpdRef : Inport
  AlphaE : Inport  Port=2
  BetaE : Inport  Port=3
  Add : Sum
  Compare To Zero1 : simulink/Logic and Bit Operations/Compare To Zero  relop=>=  OutDataTypeStr=boolean
  Constant : Constant  Value=single(200)
  Constant1 : Constant  Value=single(0.0085)
  Constant2 : Constant  Value=single(-1)
  Constant3 : Constant  Value=single(1)
  Constant4 : Constant  Value=single(10)
  Constant5 : Constant  Value=single(2*pi)
  Cos : Trigonometry  Operator=cos
  Data Type Conversion : DataTypeConversion  OutDataTypeStr=single  SaturateOnIntegerOverflow=off  RndMeth=Floor
  Data Type Conversion1 : DataTypeConversion  OutDataTypeStr=single  SaturateOnIntegerOverflow=off  RndMeth=Floor
  Delay : Delay  DelayLength=1
  Gain : Gain  Gain=0.00005
  LPF : Subsystem
  Mod : Math  Operator=mod
  PLL_PI : slpidlib/PID Controller  Controller=PI  Form=Parallel  TimeDomain=Discrete-time  UseExternalTs=off  SampleTime=-1  IntegratorMethod=Forward Euler  FilterMethod=Forward Euler  ControllerParametersSource=external  P=1  I=1  UseKiTs=on  D=0  UseExternalDerivativeSource=off  N=100  UseFilter=on  TunerSelectOption=Transfer Function Based (PID Tuner App)  InitialConditionSource=internal  InitialConditionForIntegrator=0  InitialConditionForFilter=0  DifferentiatorICPrevScaledInput=0  ExternalReset=none  TrackingMode=off  Kt=1  LimitOutput=off  SatLimitsSource=internal  UpperSaturationLimit=inf  LowerSaturationLimit=-inf  LinearizeAsGain=off  AntiWindupMode=none  Kb=1  LimitIntegrator=off  UpperIntegratorSaturationLimit=inf  LowerIntegratorSaturationLimit=-inf  POutMin=[]  POutMax=[]  IOutMin=[]  IOutMax=[]  DOutMin=[]  DOutMax=[]  NOutMin=[]  NOutMax=[]  SumOutMin=[]  SumOutMax=[]  SaturationOutMin=[]  SaturationOutMax=[]  PParamMin=[]  PParamMax=[]  IParamMin=[]  IParamMax=[]  DParamMin=[]  DParamMax=[]  NParamMin=[]  NParamMax=[]  KbParamMin=[]  KbParamMax=[]  KtParamMin=[]  KtParamMax=[]  KbOutMin=[]  KbOutMax=[]  KtOutMin=[]  KtOutMax=[]  IntegratorOutMin=[]  IntegratorOutMax=[]  FilterOutMin=[]  FilterOutMax=[]  SumI1OutMin=[]  SumI1OutMax=[]  SumI2OutMin=[]  SumI2OutMax=[]  SumI3OutMin=[]  SumI3OutMax=[]  SumI4OutMin=[]  SumI4OutMax=[]  SumDOutMin=[]  SumDOutMax=[]  DifferentiatorOutMin=[]  DifferentiatorOutMax=[]  FilterDiffOutCoefMin=[]  FilterDiffOutCoefMax=[]  ReciprocalOutMin=[]  ReciprocalOutMax=[]  SumDenOutMin=[]  SumDenOutMax=[]  SumNumOutMin=[]  SumNumOutMax=[]  DivideOutMin=[]  DivideOutMax=[]  UdiffTsProdOutMin=[]  UdiffTsProdOutMax=[]  NTsProdOutMin=[]  NTsProdOutMax=[]  UintegralTsProdOutMin=[]  UintegralTsProdOutMax=[]  UngainTsProdOutMin=[]  UngainTsProdOutMax=[]  ClampingZeroOutDataTypeStr=Inherit: Inherit via back propagation  ClampingZeroOutMin=[]  ClampingZeroOutMax=[]  FilterDenConstantOutDataTypeStr=Inherit: Inherit via back propagation  FilterDenConstantOutMin=[]  FilterDenConstantOutMax=[]  PCopyOutDataTypeStr=Inherit: Inherit via back propagation  PCopyOutMin=[]  PCopyOutMax=[]  NCopyOutDataTypeStr=Inherit: Inherit via back propagation  NCopyOutMin=[]  NCopyOutMax=[]  IntegratorContinuousStateAttributes=''  IntegratorStateMustResolveToSignalObject=off  IntegratorRTWStateStorageClass=Auto  FilterContinuousStateAttributes=''  FilterStateMustResolveToSignalObject=off  FilterRTWStateStorageClass=Auto  ParallelPVariant=ExternalParameters  IdealPVariant=Disabled  IVariant=ExternalParameters  DVariant=Disabled  IntegratorVariant=Discrete  SatVariant=Disabled  AWVariant=Passthrough  PCopyVariant=Disabled  TRVariant=Disabled  FdbkBlocksVariant=Forward  IdealPFdbkVariant=Disabled  SatFdbkVariant=Disabled  DerivativeFilterVariant=Disabled  NVariant=Disabled  NCopyVariant=Disabled_SignalSpec  FilterICVariant=Disabled  IntegratorICVariant=InternalICs  ExternalResetVariant=Disabled  TRSumVariant=Passthrough  SumFdbkVariant=Disabled  SumVariant=Sum_PI  TsampFilterVariant=InternalTs  TsampNgainVariant=Passthrough  TsampIntegralVariant=Disabled_SignalSpec  ExternalSaturationOutDataTypeStr=Inherit: Same as second input  DerivativeSourceVariant=Disabled  PreIntVariant=InternalPreInt
      settings: LibrarySourceBlock=simulink/Discrete/Discrete PID Controller
  Product{,1..3} (4 alike) : Product
  Sin : Trigonometry
  Switch1 : Switch  Criteria=u2 ~= 0  SaturateOnIntegerOverflow=off  InputSameDT=off
  err : Sum
  Thetae_Est : Outport
  We_Est : Outport  Port=2
  wires:
  MotorSpdRef/1 -> Compare To Zero1/1
  Compare To Zero1/1 -> Switch1/2
  Constant1/1 -> LPF/2(TiCon)
  LPF/1(out) -> We_Est/1
  Constant2/1 -> Switch1/1
  Constant3/1 -> Switch1/3
  Cos/1 -> Product/1
  Product/1 -> Product1/1
  Switch1/1 -> Product3/2, Product1/2
  Sin/1 -> Product2/1
  Product2/1 -> Product3/1
  Product1/1 -> err/1
  Product3/1 -> err/2
  err/1 -> PLL_PI/1
  Constant/1 -> PLL_PI/2
  Constant4/1 -> PLL_PI/3
  PLL_PI/1 -> Gain/1, LPF/1(In)
  Gain/1 -> Add/1
  Add/1 -> Mod/1
  Constant5/1 -> Mod/2
  Mod/1 -> Delay/1, Thetae_Est/1
  Delay/1 -> Cos/1, Sin/1, Add/2
  BetaE/1 -> Data Type Conversion1/1
  AlphaE/1 -> Data Type Conversion/1
  Data Type Conversion/1 -> Product/2
  Data Type Conversion1/1 -> Product2/2

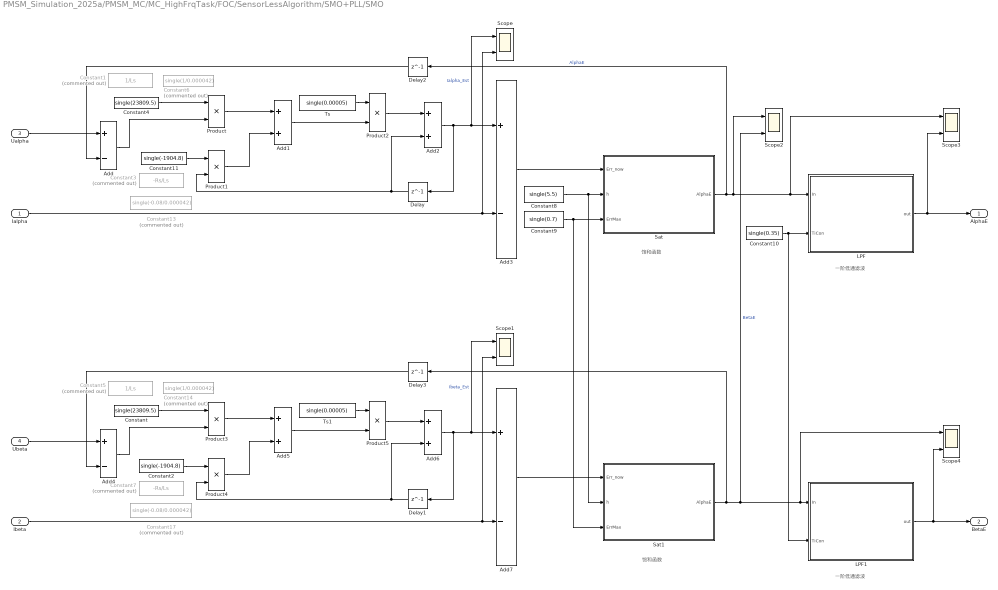
== system PMSM_Simulation_2025a/PMSM_MC/MC_HighFrqTask/FOC/SensorLessAlgorithm/SMO+PLL/SMO ==
  note: 一阶低通滤波
  note: 饱和函数
  note: 饱和函数
  note: 一阶低通滤波
  Ialpha : Inport
  Ibeta : Inport  Port=2
  Ualpha : Inport  Port=3
  Ubeta : Inport  Port=4
  Add{,3..4,7} (4 alike) : Sum  Inputs=+-
  Add{1..2,5..6} (4 alike) : Sum
  Constant : Constant  Value=single(23809.5)
  Constant1 : Constant  Commented=on  Value=1/Ls
  Constant10 : Constant  Value=single(0.35)
  Constant11 : Constant  Value=single(-1904.8)
  Constant13 : Constant  Commented=on  Value=single(-0.08/0.000042)
  Constant14 : Constant  Commented=on  Value=single(1/0.000042)
  Constant17 : Constant  Commented=on  Value=single(-0.08/0.000042)
  Constant2 : Constant  Value=single(-1904.8)
  Constant3 : Constant  Commented=on  Value=-Rs/Ls
  Constant4 : Constant  Value=single(23809.5)
  Constant5 : Constant  Commented=on  Value=1/Ls
  Constant6 : Constant  Commented=on  Value=single(1/0.000042)
  Constant7 : Constant  Commented=on  Value=-Rs/Ls
  Constant8 : Constant  Value=single(5.5)
  Constant9 : Constant  Value=single(0.7)
  Delay{,1..3} (4 alike) : Delay  DelayLength=1
  LPF : Subsystem
  LPF1 : Subsystem
  Product{,1..5} (6 alike) : Product
  Sat : Subsystem
  Sat1 : Subsystem
  Scope{,1..4} (5 alike) : Scope  NumInputPorts=2
      Scope settings: ActiveDisplayYMinimum=-11.265603890227075  ActiveDisplayYMaximum=11.401321085088421  DataLoggingVariableName=ScopeData2
      Scope1 settings: DataLoggingVariableName=ScopeData3
      Scope2 settings: ActiveDisplayYMinimum=-6.875  ActiveDisplayYMaximum=6.875  DataLoggingVariableName=ScopeData4
      Scope3 settings: DataLoggingVariableName=ScopeData5
      Scope4 settings: DataLoggingVariableName=ScopeData6
  Ts : Constant  Value=single(0.00005)
  Ts1 : Constant  Value=single(0.00005)
  AlphaE : Outport
  BetaE : Outport  Port=2
  wires:
  Ualpha/1 -> Add/1
  Constant4/1 -> Product/1
  Add/1 -> Product/2
  Product/1 -> Add1/1
  Constant11/1 -> Product1/1
  Product1/1 -> Add1/2
  Add1/1 -> Product2/2
  Ts/1 -> Product2/1
  Product2/1 -> Add2/1
  Add2/1 -> Delay/1, Scope/1, Add3/1  "Ialpha_Est"
  Delay/1 -> Add2/2, Product1/2
  Ialpha/1 -> Scope/2, Add3/2
  Product5/1 -> Add6/1
  Delay1/1 -> Add6/2, Product4/2
  Product3/1 -> Add5/1
  Ibeta/1 -> Scope1/2, Add7/2
  Ts1/1 -> Product5/1
  Add4/1 -> Product3/2
  Constant/1 -> Product3/1
  Product4/1 -> Add5/2
  Constant2/1 -> Product4/1
  Add5/1 -> Product5/2
  Add6/1 -> Delay1/1, Scope1/1, Add7/1  "Ibeta_Est"
  Ubeta/1 -> Add4/1
  Add3/1 -> Sat/1(Err_now)
  Constant8/1 -> Sat1/2(h), Sat/2(h)
  Constant9/1 -> Sat1/3(ErrMax), Sat/3(ErrMax)
  Add7/1 -> Sat1/1(Err_now)
  Sat/1(AlphaE) -> Scope2/1, Scope3/1, LPF/1(In), Delay2/1  "AlphaE"
  Delay2/1 -> Add/2
  Sat1/1(AlphaE) -> Scope2/2, Scope4/1, LPF1/1(In), Delay3/1  "BetaE"
  Delay3/1 -> Add4/2
  Constant10/1 -> LPF/2(TiCon), LPF1/2(TiCon)
  LPF/1(out) -> Scope3/2, AlphaE/1
  LPF1/1(out) -> Scope4/2, BetaE/1

== system PMSM_Simulation_2025a/PMSM_MC/MC_HighFrqTask/FOC/SensorLessAlgorithm/FluxObs+PLL/PLL/LPF ==
  In : Inport
  TiCon : Inport  Port=2
  Add : Sum  Inputs=+-
  Add1 : Sum
  Constant : Constant  Value=single(1)
  Delay : Delay  DelayLength=1  InitialConditionSource=Input port
      settings: InputPortMap=u0,p4
  Product : Product
  Product1 : Product
  out : Outport
  wires:
  Delay/1 -> Product1/2
  Add1/1 -> out/1, Delay/1
  Product1/1 -> Add1/2
  Product/1 -> Add1/1
  Constant/1 -> Add/1
  Add/1 -> Product1/1
  TiCon/1 -> Product/2, Add/2
  In/1 -> Product/1, Delay/2

== system PMSM_Simulation_2025a/PMSM_MC/MC_HighFrqTask/FOC/SensorLessAlgorithm/Luenberger+PLL/Luenberger/LPF ==
  In : Inport
  TiCon : Inport  Port=2
  Add : Sum  Inputs=+-
  Add1 : Sum
  Constant : Constant  Value=single(1)
  Delay : Delay  DelayLength=1  InitialConditionSource=Input port
      settings: InputPortMap=u0,p4
  Product : Product
  Product1 : Product
  out : Outport
  wires:
  Delay/1 -> Product1/2
  Add1/1 -> out/1, Delay/1
  Product1/1 -> Add1/2
  Product/1 -> Add1/1
  Constant/1 -> Add/1
  Add/1 -> Product1/1
  TiCon/1 -> Product/2, Add/2
  In/1 -> Product/1, Delay/2

== system PMSM_Simulation_2025a/PMSM_MC/MC_HighFrqTask/FOC/SensorLessAlgorithm/Luenberger+PLL/Luenberger/LPF1 ==
  In : Inport
  TiCon : Inport  Port=2
  Add : Sum  Inputs=+-
  Add1 : Sum
  Constant : Constant  Value=single(1)
  Delay : Delay  DelayLength=1  InitialConditionSource=Input port
      settings: InputPortMap=u0,p4
  Product : Product
  Product1 : Product
  out : Outport
  wires:
  In/1 -> Delay/2, Product/1
  TiCon/1 -> Add/2, Product/2
  Add/1 -> Product1/1
  Constant/1 -> Add/1
  Product/1 -> Add1/1
  Product1/1 -> Add1/2
  Add1/1 -> Delay/1, out/1
  Delay/1 -> Product1/2

== system PMSM_Simulation_2025a/PMSM_MC/MC_HighFrqTask/FOC/SensorLessAlgorithm/Luenberger+PLL/PLL/LPF ==
  In : Inport
  TiCon : Inport  Port=2
  Add : Sum  Inputs=+-
  Add1 : Sum
  Constant : Constant  Value=single(1)
  Delay : Delay  DelayLength=1  InitialConditionSource=Input port
      settings: InputPortMap=u0,p4
  Product : Product
  Product1 : Product
  out : Outport
  wires:
  In/1 -> Delay/2, Product/1
  TiCon/1 -> Add/2, Product/2
  Add/1 -> Product1/1
  Constant/1 -> Add/1
  Product/1 -> Add1/1
  Product1/1 -> Add1/2
  Add1/1 -> Delay/1, out/1
  Delay/1 -> Product1/2

== system PMSM_Simulation_2025a/PMSM_MC/MC_HighFrqTask/FOC/SensorLessAlgorithm/SMO+Artan/Artan/LPF ==
  In : Inport
  TiCon : Inport  Port=2
  Add : Sum  Inputs=+-
  Add1 : Sum
  Constant : Constant  Value=single(1)
  Delay : Delay  DelayLength=1  InitialConditionSource=Input port
      settings: InputPortMap=u0,p4
  Product : Product
  Product1 : Product
  out : Outport
  wires:
  In/1 -> Delay/2, Product/1
  TiCon/1 -> Add/2, Product/2
  Add/1 -> Product1/1
  Constant/1 -> Add/1
  Product/1 -> Add1/1
  Product1/1 -> Add1/2
  Add1/1 -> Delay/1, out/1
  Delay/1 -> Product1/2

== system PMSM_Simulation_2025a/PMSM_MC/MC_HighFrqTask/FOC/SensorLessAlgorithm/SMO+Artan/Artan/WeCal ==
  ArTan_theta_est : Inport
  Add{,1..2,4..5} (5 alike) : Sum  Inputs=+-
  Add3 : Sum
  Add6 : Sum
  Compare To Constant : simulink/Logic and Bit Operations/Compare To Constant  relop=<  const=-3  OutDataTypeStr=boolean
  Compare To Constant1 : simulink/Logic and Bit Operations/Compare To Constant  relop=>  const=3  OutDataTypeStr=boolean
  Constant : Constant  Value=single(0)
  Constant1 : Constant  Value=single(2*pi)
  Constant2 : Constant  Value=single(0)
  Constant3 : Constant  Value=single(2*pi)
  Delay : Delay  DelayLength=1  InitialConditionSource=Input port
      settings: InputPortMap=u0,p4
  Divide : Product  Inputs=*/
  Gain : Gain  Gain=-1
  Switch : Switch  Criteria=u2 ~= 0  SaturateOnIntegerOverflow=off  InputSameDT=off
  Switch1 : Switch  Criteria=u2 ~= 0  SaturateOnIntegerOverflow=off  InputSameDT=off
  Ts : Constant  Value=single(0.00005)
  We : Outport
  wires:
  ArTan_theta_est/1 -> Add1/1, Add/1, Delay/1, Add5/2, Delay/2
  Delay/1 -> Add4/1, Add2/2, Add/2
  Compare To Constant/1 -> Switch/2
  Add/1 -> Switch1/3, Compare To Constant1/1, Compare To Constant/1
  Constant/1 -> Add1/2
  Add1/1 -> Add3/1
  Add2/1 -> Add3/2
  Constant1/1 -> Add2/1
  Add3/1 -> Switch/1
  Constant2/1 -> Add4/2
  Constant3/1 -> Add5/1
  Add4/1 -> Add6/1
  Add5/1 -> Add6/2
  Add6/1 -> Gain/1
  Gain/1 -> Switch1/1
  Compare To Constant1/1 -> Switch1/2
  Switch1/1 -> Switch/3
  Switch/1 -> Divide/1
  Ts/1 -> Divide/2
  Divide/1 -> We/1

== system PMSM_Simulation_2025a/PMSM_MC/MC_HighFrqTask/FOC/SensorLessAlgorithm/SMO+Artan/SMO/LPF ==
  In : Inport
  TiCon : Inport  Port=2
  Add : Sum  Inputs=+-
  Add1 : Sum
  Constant : Constant  Value=single(1)
  Delay : Delay  DelayLength=1  InitialConditionSource=Input port
      settings: InputPortMap=u0,p4
  Product : Product
  Product1 : Product
  out : Outport
  wires:
  In/1 -> Delay/2, Product/1
  TiCon/1 -> Add/2, Product/2
  Add/1 -> Product1/1
  Constant/1 -> Add/1
  Product/1 -> Add1/1
  Product1/1 -> Add1/2
  Add1/1 -> Delay/1, out/1
  Delay/1 -> Product1/2
